simulink subsystem "Swerve_Odometry_sub"  (R2023b)
settings: Solver=VariableStepAuto  StartTime=0.0  StopTime=10.0  RelTol=1e-3
undefined symbols (not defined in the file): DiscIntNeverNeededParam, Motor_Rev_to_Wheel_Distance, Odometry_Reset_IC, Odometry_X_Y_TEAR, Rotation_Local_Inv
libraries: simulink x8, simulink_extras x4
settings Model: Creator=USER  LastModifiedBy=ander

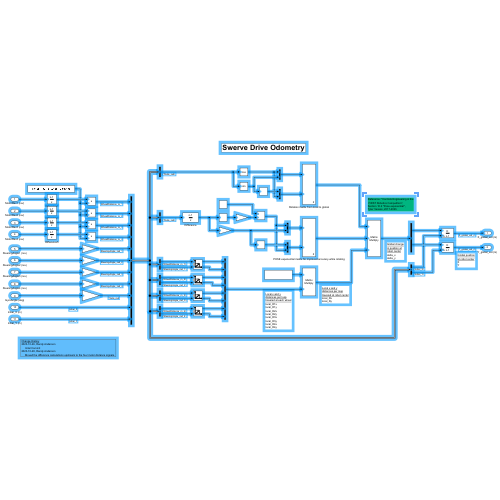
[thumbnail: Simulink's stored preview of the top-level diagram]
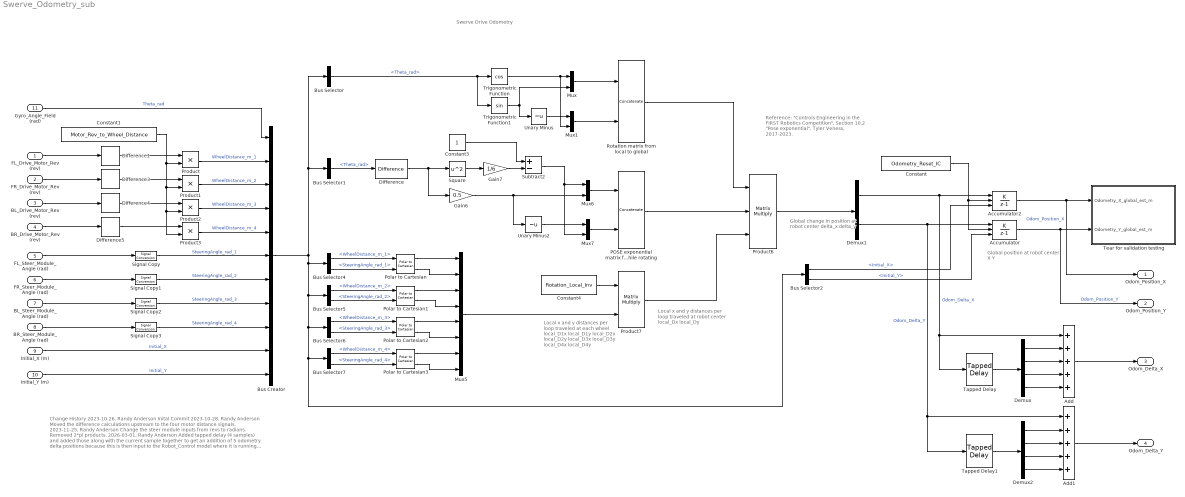
== system Swerve_Odometry_sub ==
  note: Global change
      | in position at
      | robot center
      | delta_x
      | delta_y
  note: Change History
      | 2023-10-26, Randy Anderson
      | Inital Commit
      | 2023-10-28, Randy Anderson
      | Moved the difference calculations upstream to the four motor distance signals.
      | 2023-11-25, Randy Anderson
      | Change the steer module inputs from revs to radians. Removed 2*pi products.
      | 2026-03-01, Randy Anderson
      | Added tapped delay (4 samples) and added those along with the current sample
      | together to get an addition of 5 odometry delta positions because this is then
      | input to the Robot_Control model where it is running on a 5x slower sample
      | time (20 vs. 4 msec). The output from this needs to be the total odometry
      | delta seen over the full 20 msec period.
  note: Local x and y
      | distances per loop
      | traveled at each wheel
      | local_D1x
      | local_D1y
      | local_D2x
      | local_D2y
      | local_D3x
      | local_D3y
      | local_D4x
      | local_D4y
  note: Local x and y
      | distances per loop
      | traveled at robot center
      | local_Dx
      | local_Dy
  note: Swerve Drive Odometry
  note: Global position
      | at robot center
      | X
      | Y
  note: Reference: "Controls Engineering in the
      |  FIRST Robotics Competition",
      | Section 10.2 "Pose exponential",
      | Tyler Veness, 2017-2023.
  FL_Drive_Motor_Rev (rev) : Inport
  FR_Drive_Motor_Rev (rev) : Inport  Port=2
  BL_Drive_Motor_Rev (rev) : Inport  Port=3
  BR_Drive_Motor_Rev (rev) : Inport  Port=4
  FL_Steer_Module_Angle (rad) : Inport  Port=5
  FR_Steer_Module_Angle (rad) : Inport  Port=6
  BL_Steer_Module_Angle (rad) : Inport  Port=7
  BR_Steer_Module_Angle (rad) : Inport  Port=8
  Initial_X (m) : Inport  Port=9
  Initial_Y (m) : Inport  Port=10
  Gyro_Angle_Field (rad) : Inport  Port=11
  Accumulator : DiscreteIntegrator  IntegratorMethod=Accumulation: Forward Euler  ExternalReset=rising  InitialConditionSource=external  SampleTime=-1  ICPrevOutput=DiscIntNeverNeededParam  ICPrevScaledInput=DiscIntNeverNeededParam
  Accumulator2 : DiscreteIntegrator  IntegratorMethod=Accumulation: Forward Euler  ExternalReset=rising  InitialConditionSource=external  SampleTime=-1  ICPrevOutput=DiscIntNeverNeededParam  ICPrevScaledInput=DiscIntNeverNeededParam
  Add : Sum  Inputs=5
  Add1 : Sum  Inputs=5
  Bus Creator : BusCreator  Inputs=11
  Bus Selector : BusSelector  OutputSignals=Theta_rad
  Bus Selector1 : BusSelector  OutputSignals=Theta_rad
  Bus Selector2 : BusSelector  OutputSignals=Initial_X,Initial_Y
  Bus Selector4 : BusSelector  OutputSignals=WheelDistance_m_1,SteeringAngle_rad_1
  Bus Selector5 : BusSelector  OutputSignals=WheelDistance_m_2,SteeringAngle_rad_2
  Bus Selector6 : BusSelector  OutputSignals=WheelDistance_m_3,SteeringAngle_rad_3
  Bus Selector7 : BusSelector  OutputSignals=WheelDistance_m_4,SteeringAngle_rad_4
  Constant : Constant  Value=Odometry_Reset_IC
  Constant1 : Constant  Value=Motor_Rev_to_Wheel_Distance
  Constant3 : Constant
  Constant4 : Constant  Value=Rotation_Local_Inv
  Demux : Demux
  Demux1 : Demux  Outputs=2
  Demux2 : Demux
  Difference{,1,3..5} (5 alike) : simulink/Discrete/Difference  ICPrevInput=0.0  OutMin=[]  OutMax=[]  OutDataType=fixdt(1, 16)  OutScaling=2^-10  DoSatur=off
  Gain6 : Gain  Gain=0.5
  Gain7 : Gain  Gain=1/6
  Mux{,1,6..7} (4 alike) : Mux  Inputs=2
  Mux5 : Mux  Inputs=8
  POSE exponential matrix for improved accuracy while rotating : Concatenate  Mode=Multidimensional array  ConcatenateDimension=2
  Polar to Cartesian{,1..3} (4 alike) : simulink_extras/Transformations/Polar to Cartesian
  Product{,1..3} (4 alike) : Product
  Product6 : Product  Inputs=3  Multiplication=Matrix(*)
  Product7 : Product  Multiplication=Matrix(*)
  Rotation matrix from local to global : Concatenate  Mode=Multidimensional array  ConcatenateDimension=2
  Signal Copy{,1..3} (4 alike) : SignalConversion  OverrideOpt=off
  Square : Math  Operator=square
  Subtract2 : Sum  Inputs=+-
  Tapped Delay : simulink/Discrete/Tapped Delay  vinit=0.0  samptime=-1  NumDelays=4  DelayOrder=Oldest  includeCurrent=off
  Tapped Delay1 : simulink/Discrete/Tapped Delay  vinit=0.0  samptime=-1  NumDelays=4  DelayOrder=Oldest  includeCurrent=off
  Tear for validation testing : Subsystem
  Trigonometric Function : Trigonometry  Operator=cos
  Trigonometric Function1 : Trigonometry
  Unary Minus : UnaryMinus
  Unary Minus2 : UnaryMinus
  Odom_Position_X : Outport
  Odom_Position_Y : Outport  Port=2
  Odom_Delta_X : Outport  Port=3
  Odom_Delta_Y : Outport  Port=4
  wires:
  Gain6/1 -> Mux6/2, Unary Minus2/1
  Difference5/1 -> Product3/1
  Accumulator/1 -> Tear for validation testing/2(Odometry_Y_global_est_m), Odom_Position_Y/1  "Odom_Position_Y"
  Unary Minus/1 -> Mux1/1
  Difference4/1 -> Product2/1
  BL_Drive_Motor_Rev (rev)/1 -> Difference4/1
  Difference3/1 -> Product1/1
  Unary Minus2/1 -> Mux7/1
  Subtract2/1 -> Mux7/2, Mux6/1
  Demux1/2 -> Accumulator/1, Tapped Delay1/1, Add1/1  "Odom_Delta_Y"
  Initial_Y (m)/1 -> Bus Creator/11  "Initial_Y"
  Bus Selector2/2 -> Accumulator/3  "<Initial_Y>"
  Polar to Cartesian1/1 -> Mux5/3
  Difference1/1 -> Product/1
  Bus Selector2/1 -> Accumulator2/3  "<Initial_X>"
  Product6/1 -> Demux1/1
  Polar to Cartesian3/1 -> Mux5/7
  Constant3/1 -> Subtract2/1
  Bus Selector6/2 -> Polar to Cartesian2/2  "<SteeringAngle_rad_3>"
  FR_Drive_Motor_Rev (rev)/1 -> Difference3/1
  Constant4/1 -> Product7/1
  Polar to Cartesian/2 -> Mux5/2
  Accumulator2/1 -> Tear for validation testing/1(Odometry_X_global_est_m), Odom_Position_X/1  "Odom_Position_X"
  Mux1/1 -> Rotation matrix from local to global/2
  Square/1 -> Gain7/1
  Bus Selector4/2 -> Polar to Cartesian/2  "<SteeringAngle_rad_1>"
  Bus Selector7/1 -> Polar to Cartesian3/1  "<WheelDistance_m_4>"
  Bus Selector1/1 -> Difference/1  "<Theta_rad>"
  Polar to Cartesian1/2 -> Mux5/4
  Bus Selector6/1 -> Polar to Cartesian2/1  "<WheelDistance_m_3>"
  Mux/1 -> Rotation matrix from local to global/1
  Difference/1 -> Square/1, Gain6/1
  Polar to Cartesian2/1 -> Mux5/5
  Mux5/1 -> Product7/2
  Gain7/1 -> Subtract2/2
  POSE exponential matrix for improved accuracy while rotating/1 -> Product6/2
  Mux6/1 -> POSE exponential matrix for improved accuracy while rotating/1
  Polar to Cartesian2/2 -> Mux5/6
  Product1/1 -> Bus Creator/3  "WheelDistance_m_2"
  Polar to Cartesian3/2 -> Mux5/8
  Bus Selector7/2 -> Polar to Cartesian3/2  "<SteeringAngle_rad_4>"
  Constant1/1 -> Product3/2, Product2/2, Product1/2, Product/2
  Mux7/1 -> POSE exponential matrix for improved accuracy while rotating/2
  Bus Selector/1 -> Trigonometric Function1/1, Trigonometric Function/1  "<Theta_rad>"
  Bus Selector4/1 -> Polar to Cartesian/1  "<WheelDistance_m_1>"
  Bus Selector5/2 -> Polar to Cartesian1/2  "<SteeringAngle_rad_2>"
  Gyro_Angle_Field (rad)/1 -> Bus Creator/1  "Theta_rad"
  Bus Creator/1 -> Bus Selector2/1, Bus Selector7/1, Bus Selector6/1, Bus Selector5/1, Bus Selector4/1, Bus Selector/1, Bus Selector1/1
  Trigonometric Function/1 -> Mux1/2, Mux/1
  Product7/1 -> Product6/3
  Initial_X (m)/1 -> Bus Creator/10  "Initial_X"
  Polar to Cartesian/1 -> Mux5/1
  FL_Drive_Motor_Rev (rev)/1 -> Difference1/1
  BR_Drive_Motor_Rev (rev)/1 -> Difference5/1
  Rotation matrix from local to global/1 -> Product6/1
  Product3/1 -> Bus Creator/5  "WheelDistance_m_4"
  Product/1 -> Bus Creator/2  "WheelDistance_m_1"
  Trigonometric Function1/1 -> Unary Minus/1, Mux/2
  Product2/1 -> Bus Creator/4  "WheelDistance_m_3"
  Demux1/1 -> Accumulator2/1, Tapped Delay/1, Add/1  "Odom_Delta_X"
  Bus Selector5/1 -> Polar to Cartesian1/1  "<WheelDistance_m_2>"
  FL_Steer_Module_Angle (rad)/1 -> Signal Copy/1
  FR_Steer_Module_Angle (rad)/1 -> Signal Copy1/1
  BL_Steer_Module_Angle (rad)/1 -> Signal Copy2/1
  BR_Steer_Module_Angle (rad)/1 -> Signal Copy3/1
  Signal Copy/1 -> Bus Creator/6  "SteeringAngle_rad_1"
  Signal Copy1/1 -> Bus Creator/7  "SteeringAngle_rad_2"
  Signal Copy2/1 -> Bus Creator/8  "SteeringAngle_rad_3"
  Signal Copy3/1 -> Bus Creator/9  "SteeringAngle_rad_4"
  Constant/1 -> Accumulator2/2, Accumulator/2
  Tapped Delay/1 -> Demux/1
  Demux/1 -> Add/2
  Demux/2 -> Add/3
  Demux/3 -> Add/4
  Demux/4 -> Add/5
  Tapped Delay1/1 -> Demux2/1
  Demux2/3 -> Add1/4
  Demux2/4 -> Add1/5
  Demux2/2 -> Add1/3
  Demux2/1 -> Add1/2
  Add/1 -> Odom_Delta_X/1
  Add1/1 -> Odom_Delta_Y/1

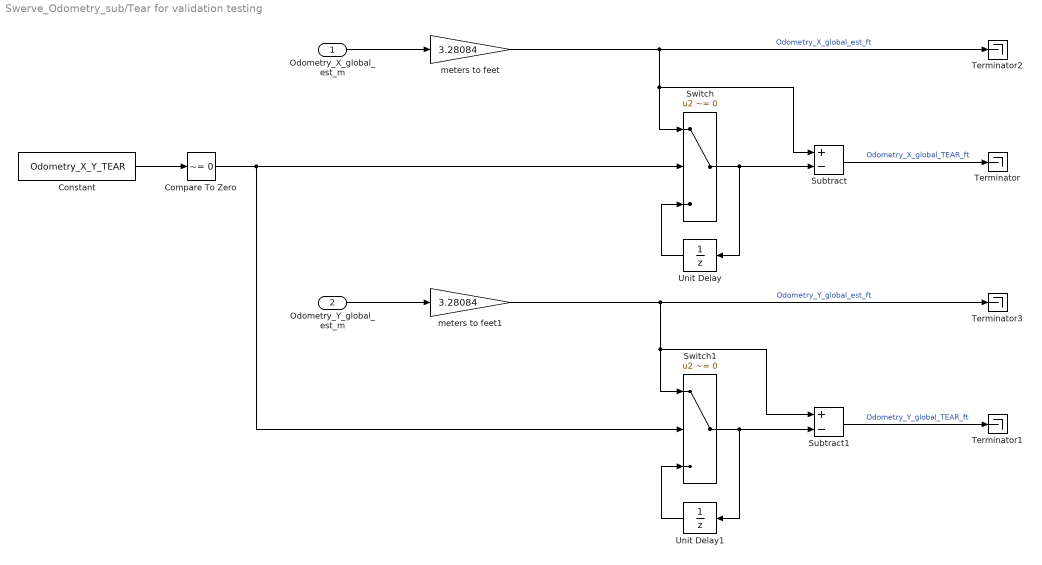
== system Swerve_Odometry_sub/Tear for validation testing ==
  Odometry_X_global_est_m : Inport
  Odometry_Y_global_est_m : Inport  Port=2
  Compare To Zero : simulink/Logic and Bit Operations/Compare To Zero  relop=~=  OutDataTypeStr=boolean
  Constant : Constant  Value=Odometry_X_Y_TEAR  OutDataTypeStr=double
  Subtract : Sum  Inputs=+-
  Subtract1 : Sum  Inputs=+-
  Switch : Switch  Criteria=u2 ~= 0  SaturateOnIntegerOverflow=off  InputSameDT=off
  Switch1 : Switch  Criteria=u2 ~= 0  SaturateOnIntegerOverflow=off  InputSameDT=off
  Terminator{,1..3} (4 alike) : Terminator
  Unit Delay : UnitDelay  SampleTime=-1  HasFrameUpgradeWarning=on
  Unit Delay1 : UnitDelay  SampleTime=-1  HasFrameUpgradeWarning=on
  meters to feet : Gain  Gain=3.28084
  meters to feet1 : Gain  Gain=3.28084
  wires:
  Compare To Zero/1 -> Switch/2, Switch1/2
  meters to feet1/1 -> Terminator3/1, Switch1/1, Subtract1/1  "Odometry_Y_global_est_ft"
  Odometry_Y_global_est_m/1 -> meters to feet1/1
  meters to feet/1 -> Subtract/1, Switch/1, Terminator2/1  "Odometry_X_global_est_ft"
  Switch1/1 -> Unit Delay1/1, Subtract1/2
  Unit Delay1/1 -> Switch1/3
  Subtract1/1 -> Terminator1/1  "Odometry_Y_global_TEAR_ft"
  Subtract/1 -> Terminator/1  "Odometry_X_global_TEAR_ft"
  Odometry_X_global_est_m/1 -> meters to feet/1
  Unit Delay/1 -> Switch/3
  Switch/1 -> Unit Delay/1, Subtract/2
  Constant/1 -> Compare To Zero/1
